simulink library "T2_Stateflow"  (R2026a)
settings: Solver=ode45  AbsTol=1e-6
undefined symbols (not defined in the file): ABS_off, ABS_on
settings Model: FPTRunName=Active  ExtModeTrigMode=oneshot  ExtModeArmWhenConnect=off  ExtModeAutoUpdateStatusClock=off  Creator=The MathWorks, Inc.  LastModifiedBy=diyar
settings DataIOCC: SignalLoggingSaveFormat=ModelDataLogs  SignalLoggingName=logsOut
settings OptimizationCC: BooleanDataType=off  InitFltsAndDblsToZero=on  EfficientMapNaN2IntZero=off  BufferReusableBoundary=off
settings DebuggingCC: SaveWithParameterizedLinksMsg=none  UnderspecifiedInitializationDetection=Classic  CheckExecutionContextPreStartOutputMsg=on  SignalResolutionControl=TryResolveAllWithWarning  MultiTaskDSMMsg=warning  MultiTaskCondExecSysMsg=none  IntegerOverflowMsg=none  IntegerSaturationMsg=none
settings HardwareCC: ProdHWDeviceType=32-bit Generic  TargetUnknown=on
settings GRTTargetCC: TargetFcnLib=ansi_tfl_tmw.mat  CombineOutputUpdateFcns=off  GRTInterface=on

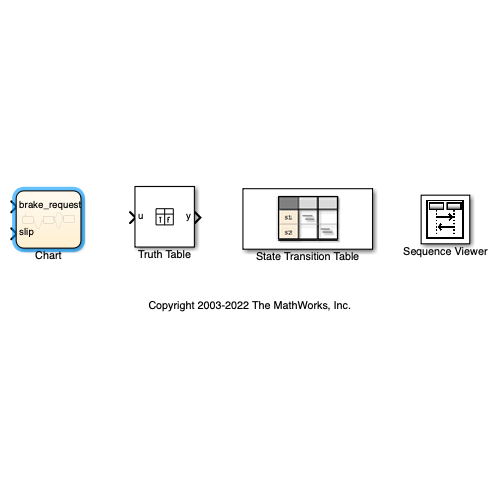
[thumbnail: Simulink's stored preview of the top-level diagram]
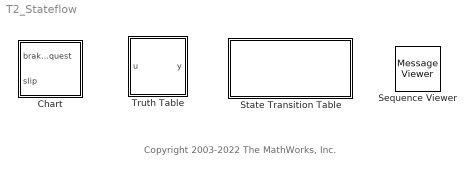
== system T2_Stateflow ==
  note: Copyright 2003-2022 The MathWorks, Inc.
  Chart : Stateflow chart  BlockKeywords=__PRM__SERIALIZED__DATA__:Stateflow Chart,Stateflow Diagram  TreatAsAtomicUnit=on
  Sequence Viewer : MessageViewer
  State Transition Table : State Transition Table  TreatAsAtomicUnit=on
  Truth Table : Truth Table  TreatAsAtomicUnit=on

== matlab function T2_Stateflow/Truth Table ==
  data: u input; y output
function y = fcn(u)

aVarTruthTableCondition_1 = false;
aVarTruthTableCondition_2 = false;


% Example condition 1

aVarTruthTableCondition_1 = logical(u >= 0);

% Example condition 2

aVarTruthTableCondition_2 = logical(u ^ 2 <= 1);

if (aVarTruthTableCondition_1 && aVarTruthTableCondition_2)
    aFcnTruthTableAction_1();
elseif (~aVarTruthTableCondition_1 && ~aVarTruthTableCondition_2)
    aFcnTruthTableAction_1();
else % Default
    aFcnTruthTableAction_2();
end

function aFcnTruthTableAction_1()

% Example action 1 called from D1 & D2 column in condition table

y = u;

function aFcnTruthTableAction_2()

% Example action 2 called from D3 column in condition table

y = 1 / u;

== stateflow chart T2_Stateflow/Chart ==
  state ABS ACTIVE
  state INACTIVE
  state BRAKING
  ABS ACTIVE -> BRAKING : [[slip <= ABS_off]]
  (default) -> INACTIVE
  BRAKING -> ABS ACTIVE : [[slip >= ABS_on]]
  INACTIVE -> BRAKING : [[brake_request == 1]]
  data: brake_request input boolean; slip input; ABS_on parameter; ABS_off parameter

== stateflow chart T2_Stateflow/State Transition Table ==
  state state1
  state state2
  (default) -> state1
  state1 -> state2
